simulink model "high_frequency_inverter_2022b_model"  (R2022b)
settings: Solver=FixedStepAuto  StartTime=0.0  StopTime=Tstop  RelTol=1e-3
values from neighbouring files (symbols this model uses):
  Cf = 0.10*(P_load/PF_ref)/(2*pi*f_out*Vout_rms^2)    (= 5.57148158972e-06)    [inverter.m]
  Co_fly = 470e-6    (= 0.00047)    [inverter.m]
  fn_tx = f_out    (= 60)    [inverter.m]
  fsw_dc = 20e3    (= 20000)    [inverter.m]
  Ipk = sqrt(2)*P_load/(Vout_rms*PF_ref)    [inverter.m]
  Ki = 0.03    [inverter.m]
  Kp = 0.002    [inverter.m]
  L1 = Vdc/(16*fsw*dI)    [inverter.m]
  L1_tx = 0.02    [inverter.m]
  L2 = L1/2    [inverter.m]
  L2_tx = 0.02    [inverter.m]
  Llk2_fly = Llk_fly*n_fly^2    (= 3.44816326531e-05)    [inverter.m]
  Llk_fly = 0.01*Lm_fly    (= 5.38775510204e-07)    [inverter.m]
  Lm_fly = Vin*D_fly/(fsw_dc*dIm)    (= 5.38775510204e-05)    [inverter.m]
  Lm_tx = 500    [inverter.m]
  m_ff = sqrt(2)*Vout_rms/Vdc    [inverter.m]
  m_max = 0.95    [inverter.m]
  m_trim = 0.1    [inverter.m]
  N_fly = round(1/(fsw_dc*Ts_power))    [inverter.m]
  PF_ref = 0.9    [inverter.m]
  Pn_fly = 1.5e3    (= 1500)    [inverter.m]
  R1_tx = 0.005    [inverter.m]
  R2_tx = 0.005    [inverter.m]
  R_d = 0.3*sqrt((L1+L2)/Cf)    [inverter.m]
  R_gnd = 1e6    (= 1000000)    [inverter.m]
  R_L1 = 0.05    [inverter.m]
  R_L2 = 0.05    [inverter.m]
  R_src = 2e-3    (= 0.002)    [inverter.m]
  Rm_fly = 10e3    (= 10000)    [inverter.m]
  Rm_tx = 500    [inverter.m]
  Rp_fly = 0.01    [inverter.m]
  Rs_fly = Rp_fly*n_fly^2    (= 0.64)    [inverter.m]
  Sn_tx = 2e3    (= 2000)    [inverter.m]
  Ts_ctrl = 1/fsw    (= 5e-05)    [inverter.m]
  Ts_power = 1/(spp*max(fsw, fsw_dc))    [inverter.m]
  V1_fly = Vin    (= 48)    [inverter.m]
  V1_tx = 230    [inverter.m]
  V2_fly = n_fly*Vin    (= 384)    [inverter.m]
  V2_tx = 230    [inverter.m]
  Vin = 48    [inverter.m]
  Vout_rms = 230    [inverter.m]
  W_fly = round(D_fly*N_fly)    [inverter.m]
  w_out = 2*pi*f_out    (= 376.991118431)    [inverter.m]
libraries: spsSeriesRLCBranchLib x7, spsVoltageMeasurementLib x6, spsCurrentMeasurementLib x4, spsGroundLib x3, spsLinearTransformerLib x2, spsRMSLib x2, spsDiodeLib x1, spsMosfetLib x1, spsMeanLib x1, spsDCVoltageSourceLib x1, spsUniversalBridgeLib x1, spsSeriesRLCLoadLib x1
settings Model: Creator=inspiredkhalid  LastModifiedBy=inspiredkhalid
settings OptimizationCC: ReuseModelBlockBuffer=on
settings RTWCC: GPUComputeCapability=5.0
settings ConfigComp: CovBoundaryAbsTol=1.0e-5

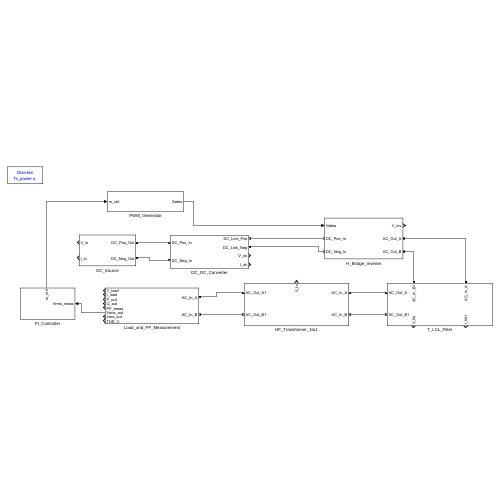
[thumbnail: Simulink's stored preview of the top-level diagram]
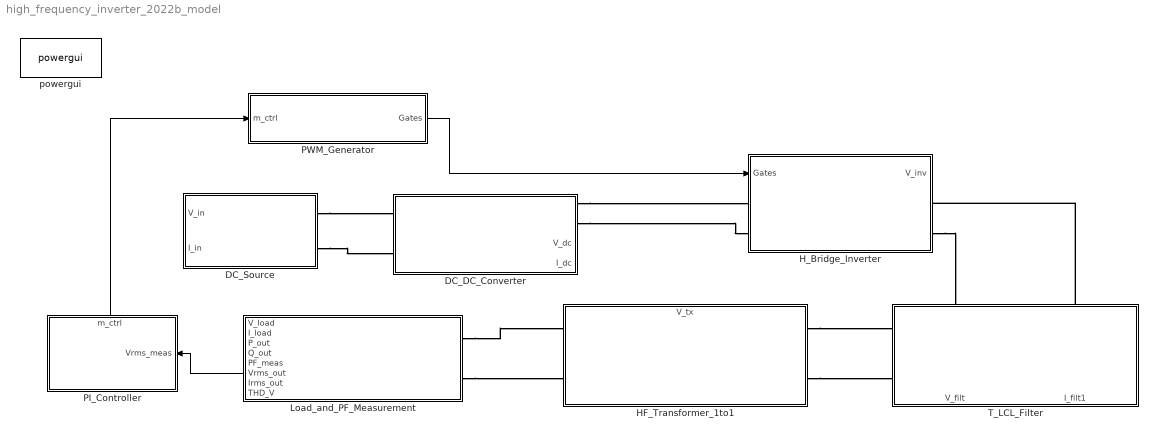
== system high_frequency_inverter_2022b_model ==
  DC_DC_Converter : Subsystem
      settings: PortSchema="{\"entries\":[{\"content\":{\"sides\":[{\"content\":{\"connectorIds\":[\"LConn1\",\"LConn2\"]},\"type\":\"ConnectorPlacement.EquallySpacedRectSide\",\"uuid\":\"edcbfbdd-8678-449a-b864-d9eb6b08d388\"},{\"content\":{\"connectorIds\":[\"RConn1\",\"RConn2\",\"Out1\",\"Out2\"],\"side\":\"RIGHT\"},\"type\":\"ConnectorPlacement.EquallySpacedRectSide\",\"uuid\":\"78ffe54f-1de1-4831-9ea2-07558472f92e\"},{\"content\":{\"side\":\"TOP\"},\"type\":\"ConnectorPlacement.EquallySpacedRectSide\",\"uuid\":\"580796b4-1520-4412-bdf9-e5b9c7a98159\"}]},\"type\":\"ConnectorPlacement.EquallySpacedConnector\",\"uuid\":\"bd2bd030-8f22-4d20-9d22-960c0cefac15\"}],\"packageUris\":[\"http://schema.mathworks.com/mf0/Connector/R2020b\"],\"version\":\"1.0\"}"
  DC_Source : Subsystem
  HF_Transformer_1to1 : Subsystem
      settings: PortSchema="{\"entries\":[{\"content\":{\"sides\":[{\"content\":{\"connectorIds\":[\"LConn1\",\"LConn2\"]},\"type\":\"ConnectorPlacement.EquallySpacedRectSide\",\"uuid\":\"99660969-c13e-4a22-bfd5-21eb4a4c8d49\"},{\"content\":{\"connectorIds\":[\"RConn1\",\"RConn2\"],\"side\":\"RIGHT\"},\"type\":\"ConnectorPlacement.EquallySpacedRectSide\",\"uuid\":\"8847538e-386e-4338-8e6c-a67f31409e40\"},{\"content\":{\"connectorIds\":[\"Out1\"],\"side\":\"TOP\"},\"type\":\"ConnectorPlacement.EquallySpacedRectSide\",\"uuid\":\"79a47430-1bd6-4e4d-bde1-bb87b2813171\"}]},\"type\":\"ConnectorPlacement.EquallySpacedConnector\",\"uuid\":\"009c51ee-68b8-4e88-a492-8a90fec86fde\"}],\"packageUris\":[\"http://schema.mathworks.com/mf0/Connector/R2020b\"],\"version\":\"1.0\"}"
  H_Bridge_Inverter : Subsystem
  Load_and_PF_Measurement : Subsystem
  PI_Controller : Subsystem
      settings: PortSchema="{\"entries\":[{\"content\":{\"sides\":[{\"content\":{\"connectorIds\":[\"In1\"]},\"type\":\"ConnectorPlacement.EquallySpacedRectSide\",\"uuid\":\"79383d80-d499-4d47-ac3d-9b177b31a5ec\"},{\"content\":{\"side\":\"RIGHT\"},\"type\":\"ConnectorPlacement.EquallySpacedRectSide\",\"uuid\":\"75656be0-e6ab-4d02-aaa1-f2d724d2565b\"},{\"content\":{\"connectorIds\":[\"Out1\"],\"side\":\"TOP\"},\"type\":\"ConnectorPlacement.EquallySpacedRectSide\",\"uuid\":\"bdbcbe30-37af-49d0-b6b4-1eafd8beb00d\"}]},\"type\":\"ConnectorPlacement.EquallySpacedConnector\",\"uuid\":\"42e5b4d1-23eb-46c2-802a-5875abd76cf7\"}],\"packageUris\":[\"http://schema.mathworks.com/mf0/Connector/R2020b\"],\"version\":\"1.0\"}"
  PWM_Generator : Subsystem
  T_LCL_Filter : Subsystem
      settings: PortSchema="{\"entries\":[{\"content\":{\"sides\":[{\"content\":{\"connectorIds\":[\"LConn1\",\"LConn2\"]},\"type\":\"ConnectorPlacement.EquallySpacedRectSide\",\"uuid\":\"edcbfbdd-8678-449a-b864-d9eb6b08d388\"},{\"content\":{\"connectorIds\":[\"Out1\",\"Out2\"],\"side\":\"RIGHT\"},\"type\":\"ConnectorPlacement.EquallySpacedRectSide\",\"uuid\":\"78ffe54f-1de1-4831-9ea2-07558472f92e\"},{\"content\":{\"connectorIds\":[\"LConn3\",\"LConn4\"],\"side\":\"TOP\"},\"type\":\"ConnectorPlacement.EquallySpacedRectSide\",\"uuid\":\"580796b4-1520-4412-bdf9-e5b9c7a98159\"}]},\"type\":\"ConnectorPlacement.EquallySpacedConnector\",\"uuid\":\"bd2bd030-8f22-4d20-9d22-960c0cefac15\"}],\"packageUris\":[\"http://schema.mathworks.com/mf0/Connector/R2020b\"],\"version\":\"1.0\"}"
  powergui : spspowerguiLib/powergui  Priority=1  SimulationMode=Discrete  SampleTime=Ts_power  frequency=f_out  Iterations=50  frequencyindice=0  Pbase=100e6  ErrMax=1e-4  UnitsV=kV  UnitsW=MW  buscounter=0  FunctionMessages=off  echomessages=off  EnableUseOfTLC=off  CurrentSourceSwitches=off  DisableSnubberDevices=off  DisableRonSwitches=off  DisableVfSwitches=off  DisplayEquations=off  AutomaticDiscreteSolvers=off  SolverType=Tustin/Backward Euler (TBE)  Interpol=off  ExternalGateDelay=off  methode=off  Ts=100  x0status=blocks  SPID=on  SwTol=0  HookPort=off  NonlinearTolerance=1e-4  nMaxIteration=100  ContinueOnMaxIteration=off  RestoreLinks=warning  ResistiveCurrentMeasurement=off  Frange=[0:2:500]  Ylog=off  Xlog=on  ShowGrid=off  save=off  variable=ZData  structure=0  ZoomFFT=off  StartTime=0.0  cycles=1  DisplayStyle=1  fundamental=60  FreqAxis=off  MaxFrequency=1000  frequencyindicesteady=1  RmsSteady=1  display=off
  wires:
  PI_Controller/1(m_ctrl) -> PWM_Generator/1(m_ctrl)
  PWM_Generator/1(Gates) -> H_Bridge_Inverter/1(Gates)
  Load_and_PF_Measurement/6(Vrms_out) -> PI_Controller/1(Vrms_meas)
  connections:
  DC_Source/LConn1 -- DC_DC_Converter/LConn1
  DC_Source/LConn2 -- DC_DC_Converter/LConn2
  DC_DC_Converter/RConn1 -- H_Bridge_Inverter/LConn1
  DC_DC_Converter/RConn2 -- H_Bridge_Inverter/LConn2
  T_LCL_Filter/LConn2 -- H_Bridge_Inverter/RConn1
  H_Bridge_Inverter/RConn2 -- T_LCL_Filter/LConn1
  HF_Transformer_1to1/RConn1 -- T_LCL_Filter/LConn3
  HF_Transformer_1to1/RConn2 -- T_LCL_Filter/LConn4
  Load_and_PF_Measurement/LConn1 -- HF_Transformer_1to1/LConn1
  Load_and_PF_Measurement/LConn2 -- HF_Transformer_1to1/LConn2

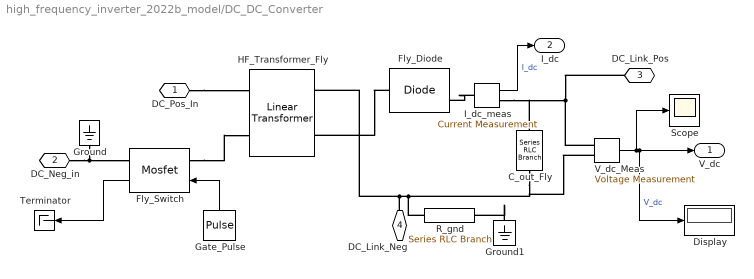
== system high_frequency_inverter_2022b_model/DC_DC_Converter ==
  C_out_Fly : spsSeriesRLCBranchLib/Series RLC Branch  LConnTagsString=__new0  RConnTagsString=__new0  BranchType=C  Resistance=1  Inductance=1e-3  SetiL0=off  InitialCurrent=0  Capacitance=Co_fly  Setx0=off  InitialVoltage=0  Measurements=None
  Display : Display
  Fly_Diode : spsDiodeLib/Diode  Ron=Rd_diode  Lon=0  Vf=Vf_diode  IC=0  UseSnubber=0  Rs=Rsn  Cs=Csn  Measurements=on
  Fly_Switch : spsMosfetLib/Mosfet  Ron=Rds_on_dc  Lon=0  Rd=Rd_diode  Vfd=Vf_diode  IC=0  Rs=Rsn  Cs=Csn  Measurements=on
  Gate_Pulse : DiscretePulseGenerator  Period=N_fly  PulseWidth=W_fly  SampleTime=Ts_power
  Ground : spsGroundLib/Ground  LConnTagsString=a
  Ground1 : spsGroundLib/Ground  LConnTagsString=a
  HF_Transformer_Fly : spsLinearTransformerLib/Linear Transformer  UNITS=SI  NominalPower=[ Pn_fly fsw_dc ]  winding1=[V1_fly Rp_fly Llk_fly]  winding2=[V2_fly Rs_fly Llk2_fly]  ThreeWindings=off  winding3=[3.15e+05 0.7938 0.084225]  RmLm=[Rm_fly Lm_fly]  Measurements=None  DataType=on
  I_dc_meas : spsCurrentMeasurementLib/Current Measurement  PhasorSimulation=off  OutputType=Complex  PSBequivalent=0
  R_gnd : spsSeriesRLCBranchLib/Series RLC Branch  LConnTagsString=__new0  RConnTagsString=__new0  BranchType=R  Resistance=R_gnd  Inductance=1e-3  SetiL0=off  InitialCurrent=0  Capacitance=1e-6  Setx0=off  InitialVoltage=0  Measurements=None
  Scope : Scope
  Terminator : Terminator
  V_dc_Meas : spsVoltageMeasurementLib/Voltage Measurement  PhasorSimulation=off  OutputType=Complex  PSBequivalent=0
  DC_Pos_In : PMIOPort  Side=Left
  DC_Neg_in : PMIOPort  Port=2  Side=Left
  DC_Link_Pos : PMIOPort  Port=3  Side=Right
  DC_Link_Neg : PMIOPort  Port=4  Side=Right
  V_dc : Outport
  I_dc : Outport  Port=2
  wires:
  Gate_Pulse/1 -> Fly_Switch/1
  Fly_Switch/1 -> Terminator/1
  V_dc_Meas/1 -> Scope/1, Display/1, V_dc/1  "V_dc"
  I_dc_meas/1 -> I_dc/1  "I_dc"
  connections:
  DC_Pos_In/RConn1 -- HF_Transformer_Fly/LConn1
  Fly_Switch/LConn1 -- HF_Transformer_Fly/LConn2
  DC_Neg_in/RConn1 -- Ground/LConn1 -- Fly_Switch/RConn1
  Fly_Diode/LConn1 -- HF_Transformer_Fly/RConn2
  DC_Link_Pos/RConn1 -- C_out_Fly/LConn1 -- I_dc_meas/RConn1 -- V_dc_Meas/LConn1
  DC_Link_Neg/RConn1 -- R_gnd/LConn1 -- C_out_Fly/RConn1 -- V_dc_Meas/LConn2 -- HF_Transformer_Fly/RConn1
  I_dc_meas/LConn1 -- Fly_Diode/RConn1
  Ground1/LConn1 -- R_gnd/RConn1

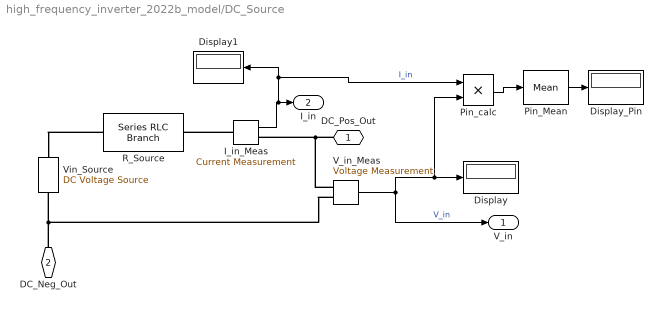
== system high_frequency_inverter_2022b_model/DC_Source ==
  Display : Display
  Display1 : Display
  Display_Pin : Display
  I_in_Meas : spsCurrentMeasurementLib/Current Measurement  PhasorSimulation=off  OutputType=Complex  PSBequivalent=0
  Pin_Mean : spsMeanLib/Mean  Freq=f_out  Vinit=0  Ts=0
  Pin_calc : Product
  R_Source : spsSeriesRLCBranchLib/Series RLC Branch  LConnTagsString=__new0  RConnTagsString=__new0  BranchType=R  Resistance=R_src  Inductance=0  SetiL0=off  InitialCurrent=0  Capacitance=inf  Setx0=off  InitialVoltage=0  Measurements=None
  V_in_Meas : spsVoltageMeasurementLib/Voltage Measurement  PhasorSimulation=off  OutputType=Complex  PSBequivalent=0
  Vin_Source : spsDCVoltageSourceLib/DC Voltage Source  Amplitude=Vin  Measurements=None
  DC_Pos_Out : PMIOPort  Side=Left
  DC_Neg_Out : PMIOPort  Port=2  Side=Left
  V_in : Outport
  I_in : Outport  Port=2
  wires:
  V_in_Meas/1 -> V_in/1, Pin_calc/2, Display/1  "V_in"
  I_in_Meas/1 -> Pin_calc/1, Display1/1, I_in/1  "I_in"
  Pin_calc/1 -> Pin_Mean/1
  Pin_Mean/1 -> Display_Pin/1
  connections:
  R_Source/LConn1 -- Vin_Source/RConn1
  I_in_Meas/LConn1 -- R_Source/RConn1
  DC_Pos_Out/RConn1 -- V_in_Meas/LConn1 -- I_in_Meas/RConn1
  DC_Neg_Out/RConn1 -- Vin_Source/LConn1 -- V_in_Meas/LConn2

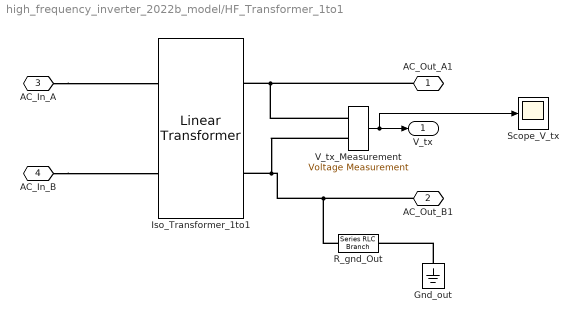
== system high_frequency_inverter_2022b_model/HF_Transformer_1to1 ==
  Gnd_out : spsGroundLib/Ground  LConnTagsString=a
  Iso_Transformer_1to1 : spsLinearTransformerLib/Linear Transformer  UNITS=pu  NominalPower=[ Sn_tx fn_tx]  winding1="[ V1_tx  R1_tx  L1_tx ]"  winding2="[V2_tx  R2_tx  L2_tx ]"  ThreeWindings=off  winding3=[ 315e3 0.002 0.08 ]  RmLm=[ Rm_tx Lm_tx ]  Measurements=None  DataType=off
  R_gnd_Out : spsSeriesRLCBranchLib/Series RLC Branch  LConnTagsString=__new0  RConnTagsString=__new0  BranchType=R  Resistance=R_gnd  Inductance=1e-3  SetiL0=off  InitialCurrent=0  Capacitance=1e-6  Setx0=off  InitialVoltage=0  Measurements=None
  Scope_V_tx : Scope
  V_tx_Measurement : spsVoltageMeasurementLib/Voltage Measurement  PhasorSimulation=off  OutputType=Complex  PSBequivalent=0
  AC_Out_A1 : PMIOPort  Side=Left
  AC_Out_B1 : PMIOPort  Port=2  Side=Left
  AC_In_A : PMIOPort  Port=3  Side=Right
  AC_In_B : PMIOPort  Port=4  Side=Right
  V_tx : Outport
  wires:
  V_tx_Measurement/1 -> Scope_V_tx/1, V_tx/1
  connections:
  AC_In_A/RConn1 -- Iso_Transformer_1to1/LConn1
  AC_In_B/RConn1 -- Iso_Transformer_1to1/LConn2
  AC_Out_A1/RConn1 -- V_tx_Measurement/LConn1 -- Iso_Transformer_1to1/RConn1
  AC_Out_B1/RConn1 -- V_tx_Measurement/LConn2 -- Iso_Transformer_1to1/RConn2 -- R_gnd_Out/LConn1
  Gnd_out/LConn1 -- R_gnd_Out/RConn1

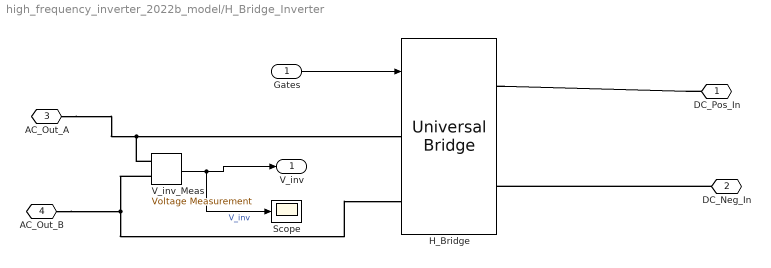
== system high_frequency_inverter_2022b_model/H_Bridge_Inverter ==
  Gates : Inport
  H_Bridge : spsUniversalBridgeLib/Universal Bridge  Arms=2  SnubberResistance=Rsn  SnubberCapacitance=Csn  Device=MOSFET / Diodes  Ron=Rds_on_inv  Lon=0  ForwardVoltages="[  0  0  ]"  ForwardVoltage=0  GTOparameters=[ 10e-6 , 20e-6 ]  IGBTparameters=[ 1e-6 , 2e-6 ]  Measurements=None  Measurements_2=None  converterType=Rectifier
  Scope : Scope
  V_inv_Meas : spsVoltageMeasurementLib/Voltage Measurement  PhasorSimulation=off  OutputType=Complex  PSBequivalent=0
  DC_Pos_In : PMIOPort  Side=Left
  DC_Neg_In : PMIOPort  Port=2  Side=Left
  AC_Out_A : PMIOPort  Port=3  Side=Right
  AC_Out_B : PMIOPort  Port=4  Side=Right
  V_inv : Outport
  wires:
  Gates/1 -> H_Bridge/1
  V_inv_Meas/1 -> Scope/1, V_inv/1  "V_inv"
  connections:
  DC_Neg_In/RConn1 -- H_Bridge/RConn2
  DC_Pos_In/RConn1 -- H_Bridge/RConn1
  AC_Out_A/RConn1 -- V_inv_Meas/LConn1 -- H_Bridge/LConn1
  AC_Out_B/RConn1 -- V_inv_Meas/LConn2 -- H_Bridge/LConn2

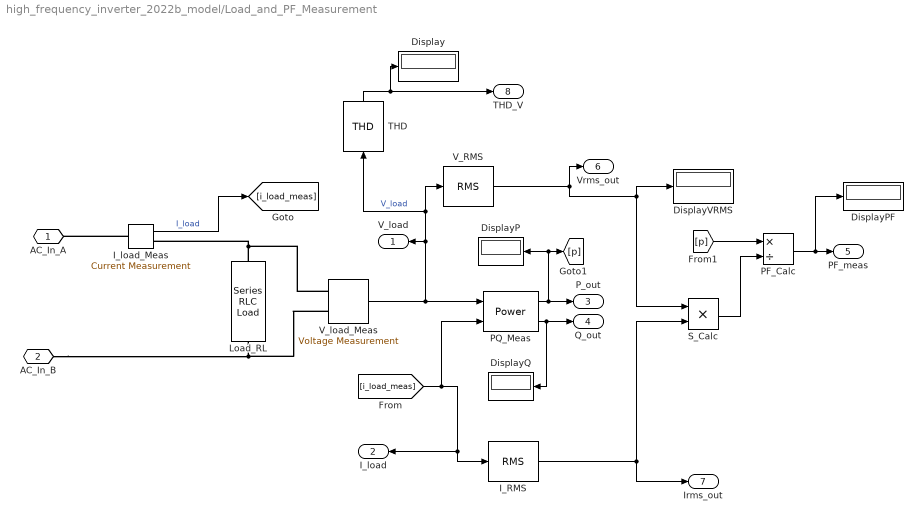
== system high_frequency_inverter_2022b_model/Load_and_PF_Measurement ==
  Display : Display
  DisplayP : Display
  DisplayPF : Display
  DisplayQ : Display
  DisplayVRMS : Display
  I_RMS : spsRMSLib/RMS  TrueRMS=on  Freq=f_out  RMSInit=120  Ts=Ts_ctrl
  I_load_Meas : spsCurrentMeasurementLib/Current Measurement  PhasorSimulation=off  OutputType=Complex  PSBequivalent=0
  "Load_RL " : spsSeriesRLCLoadLib/Series RLC Load  LConnTagsString=a  RConnTagsString=__new0  NominalVoltage=Vout_rms  NominalFrequency=f_out  ActivePower=P_load  InductivePower=Q_load  CapacitivePower=0  Setx0=off  InitialVoltage=0  SetiL0=off  InitialCurrent=0  Measurements=None  LoadType=constant Z
  PF_Calc : Product  Inputs=*/
  PQ_Meas : spsPowerLib/Power  Freq=f_out  Vinit=[sqrt(2)*Vout_rms 0]  Iinit=[Ipk -acosd(PF_ref)]  Ts=Ts_ctrl
  S_Calc : Product
  "THD " : spsTHDLib/THD  Freq=f_out  Ts=Ts_ctrl
  V_RMS : spsRMSLib/RMS  TrueRMS=on  Freq=f_out  RMSInit=120  Ts=Ts_ctrl
  V_load_Meas : spsVoltageMeasurementLib/Voltage Measurement  PhasorSimulation=off  OutputType=Complex  PSBequivalent=0
  AC_In_A : PMIOPort  Side=Left
  AC_In_B : PMIOPort  Port=2  Side=Left
  V_load : Outport
  I_load : Outport  Port=2
  P_out : Outport  Port=3
  Q_out : Outport  Port=4
  PF_meas : Outport  Port=5
  Vrms_out : Outport  Port=6
  Irms_out : Outport  Port=7
  THD_V : Outport  Port=8
  wires:
  I_load_Meas/1 -> [i_load_meas]  "I_load"
  [i_load_meas] -> I_load/1, I_RMS/1, PQ_Meas/2
  V_RMS/1 -> S_Calc/1, DisplayVRMS/1, Vrms_out/1
  I_RMS/1 -> S_Calc/2, Irms_out/1
  PQ_Meas/2 -> DisplayQ/1, Q_out/1
  S_Calc/1 -> PF_Calc/2
  PF_Calc/1 -> DisplayPF/1, PF_meas/1
  "THD "/1 -> Display/1, THD_V/1
  V_load_Meas/1 -> V_load/1, V_RMS/1, "THD "/1, PQ_Meas/1  "V_load"
  [p] -> PF_Calc/1
  PQ_Meas/1 -> DisplayP/1, [p], P_out/1
  connections:
  I_load_Meas/LConn1 -- AC_In_A/RConn1
  "Load_RL "/LConn1 -- I_load_Meas/RConn1 -- V_load_Meas/LConn1
  AC_In_B/RConn1 -- V_load_Meas/LConn2 -- "Load_RL "/RConn1

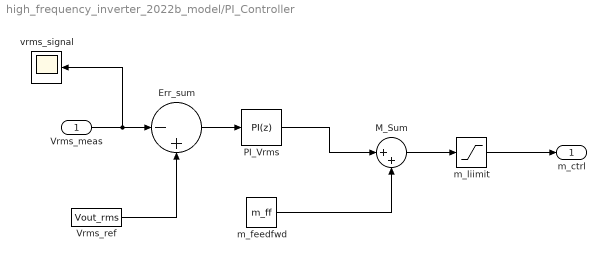
== system high_frequency_inverter_2022b_model/PI_Controller ==
  Vrms_meas : Inport
  Err_sum : Sum  Inputs=|-+
  M_Sum : Sum  Inputs=|++
  PI_Vrms : slpidlib/PID Controller  Controller=PI  Form=Parallel  TimeDomain=Discrete-time  UseExternalTs=off  SampleTime=Ts_ctrl  IntegratorMethod=Forward Euler  FilterMethod=Forward Euler  ControllerParametersSource=internal  P=Kp  I=Ki  UseKiTs=off  D=0  N=100  UseFilter=on  TunerSelectOption=Transfer Function Based (PID Tuner App)  InitialConditionSource=internal  InitialConditionForIntegrator=0  InitialConditionForFilter=0  DifferentiatorICPrevScaledInput=0  ExternalReset=none  TrackingMode=off  Kt=1  LimitOutput=on  SatLimitsSource=internal  UpperSaturationLimit=m_trim  LowerSaturationLimit=-m_trim  LinearizeAsGain=off  AntiWindupMode=clamping  Kb=1  LimitIntegrator=off  UpperIntegratorSaturationLimit=inf  LowerIntegratorSaturationLimit=-inf  POutMin=[]  POutMax=[]  IOutMin=[]  IOutMax=[]  DOutMin=[]  DOutMax=[]  NOutMin=[]  NOutMax=[]  SumOutMin=[]  SumOutMax=[]  SaturationOutMin=[]  SaturationOutMax=[]  PParamMin=[]  PParamMax=[]  IParamMin=[]  IParamMax=[]  DParamMin=[]  DParamMax=[]  NParamMin=[]  NParamMax=[]  KbParamMin=[]  KbParamMax=[]  KtParamMin=[]  KtParamMax=[]  KbOutMin=[]  KbOutMax=[]  KtOutMin=[]  KtOutMax=[]  IntegratorOutMin=[]  IntegratorOutMax=[]  FilterOutMin=[]  FilterOutMax=[]  SumI1OutMin=[]  SumI1OutMax=[]  SumI2OutMin=[]  SumI2OutMax=[]  SumI3OutMin=[]  SumI3OutMax=[]  SumI4OutMin=[]  SumI4OutMax=[]  SumDOutMin=[]  SumDOutMax=[]  DifferentiatorOutMin=[]  DifferentiatorOutMax=[]  FilterDiffOutCoefMin=[]  FilterDiffOutCoefMax=[]  ReciprocalOutMin=[]  ReciprocalOutMax=[]  SumDenOutMin=[]  SumDenOutMax=[]  SumNumOutMin=[]  SumNumOutMax=[]  DivideOutMin=[]  DivideOutMax=[]  UdiffTsProdOutMin=[]  UdiffTsProdOutMax=[]  NTsProdOutMin=[]  NTsProdOutMax=[]  UintegralTsProdOutMin=[]  UintegralTsProdOutMax=[]  UngainTsProdOutMin=[]  UngainTsProdOutMax=[]  IntegratorContinuousStateAttributes=''  IntegratorStateMustResolveToSignalObject=off  IntegratorRTWStateStorageClass=Auto  FilterContinuousStateAttributes=''  FilterStateMustResolveToSignalObject=off  FilterRTWStateStorageClass=Auto  ParallelPVariant=InternalParameters  IdealPVariant=Disabled  IVariant=InternalParameters  DVariant=Disabled  IntegratorVariant=Discrete  SatVariant=Enabled  AWVariant=DiscClampingParallel  PCopyVariant=Disabled  TRVariant=Disabled  FdbkBlocksVariant=Forward  IdealPFdbkVariant=Disabled  SatFdbkVariant=Disabled  DerivativeFilterVariant=Disabled  NVariant=Disabled  NCopyVariant=Disabled_SignalSpec  FilterICVariant=Disabled  IntegratorICVariant=InternalICs  ExternalResetVariant=Disabled  TRSumVariant=Passthrough  SumFdbkVariant=Disabled  SumVariant=Sum_PI  TsampFilterVariant=InternalTs  TsampNgainVariant=Passthrough  TsampIntegralVariant=Disabled_SignalSpec  ExternalSaturationOutDataTypeStr=Inherit: Same as second input
      settings: LibrarySourceBlock=simulink/Discrete/Discrete PID Controller
  Vrms_ref : Constant  Value=Vout_rms
  m_feedfwd : Constant  Value=m_ff
  m_liimit : Saturate  UpperLimit=m_max  LowerLimit=0
  vrms_signal : Scope
  m_ctrl : Outport
  wires:
  Vrms_meas/1 -> vrms_signal/1, Err_sum/1
  Vrms_ref/1 -> Err_sum/2
  Err_sum/1 -> PI_Vrms/1
  PI_Vrms/1 -> M_Sum/1
  m_feedfwd/1 -> M_Sum/2
  M_Sum/1 -> m_liimit/1
  m_liimit/1 -> m_ctrl/1

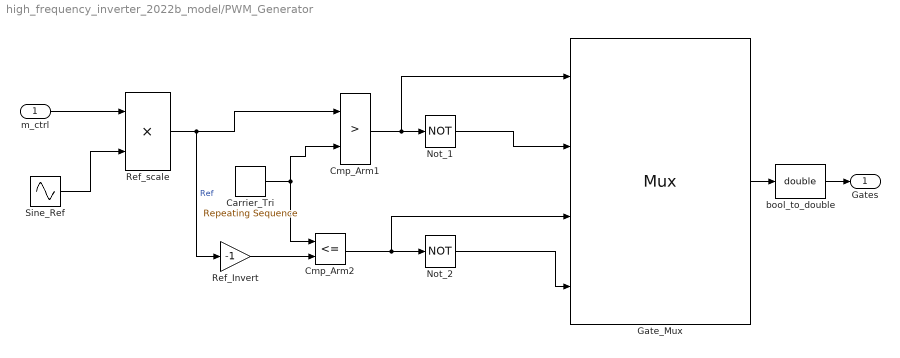
== system high_frequency_inverter_2022b_model/PWM_Generator ==
  m_ctrl : Inport
  Carrier_Tri : simulink/Sources/Repeating Sequence  rep_seq_t=t_tri  rep_seq_y=v_tri
  Cmp_Arm1 : RelationalOperator  Operator=>  OutDataTypeStr=boolean  RndMeth=Simplest  InputSameDT=off
  Cmp_Arm2 : RelationalOperator  Operator=<=  OutDataTypeStr=boolean  RndMeth=Simplest  InputSameDT=off
  Gate_Mux : Mux
  Not_1 : Logic  Operator=NOT  AllPortsSameDT=off  OutDataTypeStr=boolean
  Not_2 : Logic  Operator=NOT  AllPortsSameDT=off  OutDataTypeStr=boolean
  Ref_Invert : Gain  Gain=-1
  Ref_scale : Product
  Sine_Ref : Sin  Frequency=w_out  SampleTime=Ts_power
  bool_to_double : DataTypeConversion  OutDataTypeStr=double  SaturateOnIntegerOverflow=off  RndMeth=Floor
  Gates : Outport
  wires:
  Sine_Ref/1 -> Ref_scale/2
  m_ctrl/1 -> Ref_scale/1
  Ref_scale/1 -> Ref_Invert/1, Cmp_Arm1/1  "Ref"
  Ref_Invert/1 -> Cmp_Arm2/2
  Carrier_Tri/1 -> Cmp_Arm1/2, Cmp_Arm2/1
  Cmp_Arm2/1 -> Gate_Mux/3, Not_2/1
  Cmp_Arm1/1 -> Gate_Mux/1, Not_1/1
  Not_2/1 -> Gate_Mux/4
  Not_1/1 -> Gate_Mux/2
  Gate_Mux/1 -> bool_to_double/1
  bool_to_double/1 -> Gates/1

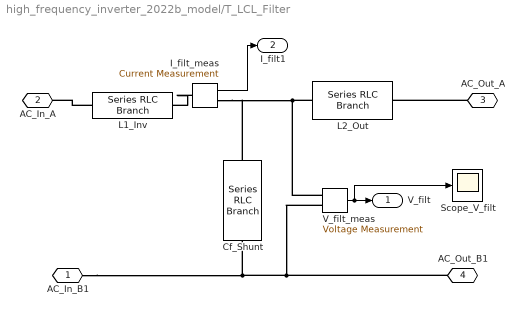
== system high_frequency_inverter_2022b_model/T_LCL_Filter ==
  Cf_Shunt : spsSeriesRLCBranchLib/Series RLC Branch  LConnTagsString=__new0  RConnTagsString=__new0  BranchType=RC  Resistance=R_d  Inductance=L2  SetiL0=off  InitialCurrent=0  Capacitance=Cf  Setx0=off  InitialVoltage=0  Measurements=None
  I_filt_meas : spsCurrentMeasurementLib/Current Measurement  PhasorSimulation=off  OutputType=Complex  PSBequivalent=0
  L1_Inv : spsSeriesRLCBranchLib/Series RLC Branch  LConnTagsString=__new0  RConnTagsString=__new0  BranchType=RL  Resistance=R_L1  Inductance=L1  SetiL0=off  InitialCurrent=0  Capacitance=1e-6  Setx0=off  InitialVoltage=0  Measurements=None
  L2_Out : spsSeriesRLCBranchLib/Series RLC Branch  LConnTagsString=__new0  RConnTagsString=__new0  BranchType=RL  Resistance=R_L2  Inductance=L2  SetiL0=off  InitialCurrent=0  Capacitance=1e-6  Setx0=off  InitialVoltage=0  Measurements=None
  Scope_V_filt : Scope
  V_filt_meas : spsVoltageMeasurementLib/Voltage Measurement  PhasorSimulation=off  OutputType=Complex  PSBequivalent=0
  AC_In_B1 : PMIOPort  Side=Left
  "AC_In_A " : PMIOPort  Port=2  Side=Left
  AC_Out_A : PMIOPort  Port=3  Side=Left
  AC_Out_B1 : PMIOPort  Port=4  Side=Left
  V_filt : Outport
  I_filt1 : Outport  Port=2
  wires:
  I_filt_meas/1 -> I_filt1/1
  V_filt_meas/1 -> Scope_V_filt/1, V_filt/1
  connections:
  L1_Inv/LConn1 -- "AC_In_A "/RConn1
  L2_Out/LConn1 -- Cf_Shunt/LConn1 -- I_filt_meas/RConn1 -- V_filt_meas/LConn1
  AC_Out_A/RConn1 -- L2_Out/RConn1
  V_filt_meas/LConn2 -- Cf_Shunt/RConn1 -- AC_In_B1/RConn1 -- AC_Out_B1/RConn1
  I_filt_meas/LConn1 -- L1_Inv/RConn1
